simulink model "ai_layered_control_bench"  (R2024b)
settings: Solver=ode1  StartTime=0.0  StopTime=40  FixedStep=0.001  RelTol=1e-3
settings Model: Creator=ai-layered-control  LastModifiedBy=xiaol

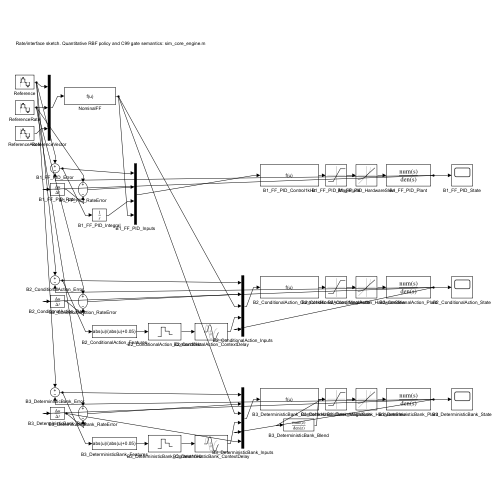
[thumbnail: Simulink's stored preview of the top-level diagram]
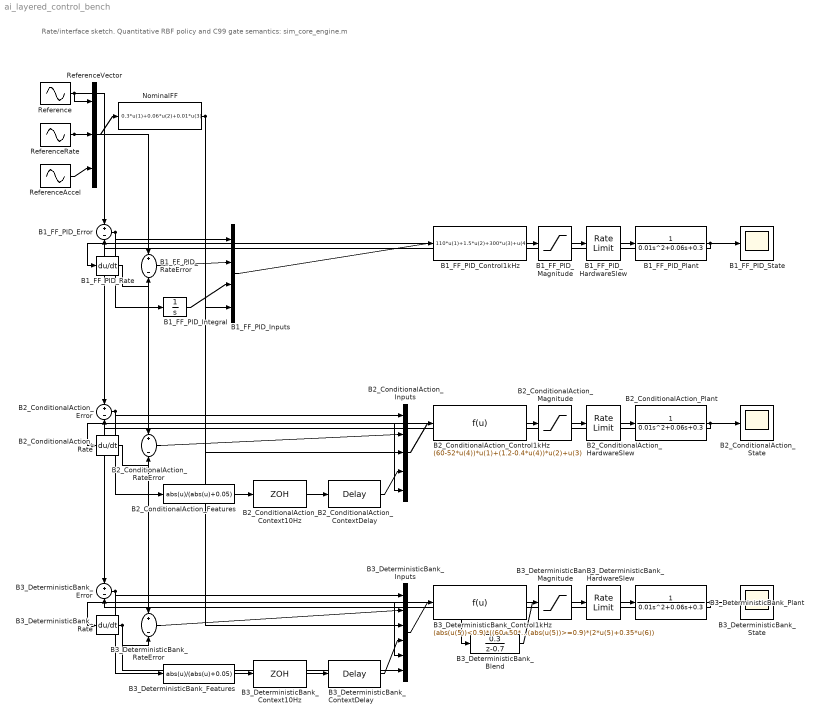
== system ai_layered_control_bench ==
  note: Rate/interface sketch. Quantitative RBF policy and C99 gate semantics: sim_core_engine.m
  B1_FF_PID_Control1kHz : Fcn  Expr=110*u(1)+1.5*u(2)+300*u(3)+u(4)
  B1_FF_PID_Error : Sum  Inputs=+-
  B1_FF_PID_HardwareSlew : RateLimiter  RisingSlewLimit=2000  FallingSlewLimit=-2000  SampleTimeMode=inherited
  B1_FF_PID_Inputs : Mux
  B1_FF_PID_Integral : Integrator
  B1_FF_PID_Magnitude : Saturate  UpperLimit=20  LowerLimit=-20
  B1_FF_PID_Plant : TransferFcn  Denominator=[0.01 0.06 0.3]
  B1_FF_PID_Rate : Derivative
  B1_FF_PID_RateError : Sum  Inputs=+-
  B1_FF_PID_State : Scope
  B2_ConditionalAction_Context10Hz : ZeroOrderHold  SampleTime=0.1
  B2_ConditionalAction_ContextDelay : TransportDelay  DelayTime=0.1
  B2_ConditionalAction_Control1kHz : Fcn  Expr=(60-52*u(4))*u(1)+(1.2-0.4*u(4))*u(2)+u(3)
  B2_ConditionalAction_Error : Sum  Inputs=+-
  B2_ConditionalAction_Features : Fcn  Expr=abs(u)/(abs(u)+0.05)
  B2_ConditionalAction_HardwareSlew : RateLimiter  RisingSlewLimit=2000  FallingSlewLimit=-2000  SampleTimeMode=inherited
  B2_ConditionalAction_Inputs : Mux  Inputs=5
  B2_ConditionalAction_Magnitude : Saturate  UpperLimit=20  LowerLimit=-20
  B2_ConditionalAction_Plant : TransferFcn  Denominator=[0.01 0.06 0.3]
  B2_ConditionalAction_Rate : Derivative
  B2_ConditionalAction_RateError : Sum  Inputs=+-
  B2_ConditionalAction_State : Scope
  B3_DeterministicBank_Blend : DiscreteTransferFcn  Numerator=[0.3]  Denominator=[1 -0.7]  SampleTime=0.001
  B3_DeterministicBank_Context10Hz : ZeroOrderHold  SampleTime=0.1
  B3_DeterministicBank_ContextDelay : TransportDelay  DelayTime=0.1
  B3_DeterministicBank_Control1kHz : Fcn  Expr=(abs(u(5))<0.9)*((60+50*(u(4)>0.5))*u(1)+1.2*u(2)+u(3))-(abs(u(5))>=0.9)*(2*u(5)+0.35*u(6))
  B3_DeterministicBank_Error : Sum  Inputs=+-
  B3_DeterministicBank_Features : Fcn  Expr=abs(u)/(abs(u)+0.05)
  B3_DeterministicBank_HardwareSlew : RateLimiter  RisingSlewLimit=2000  FallingSlewLimit=-2000  SampleTimeMode=inherited
  B3_DeterministicBank_Inputs : Mux  Inputs=6
  B3_DeterministicBank_Magnitude : Saturate  UpperLimit=20  LowerLimit=-20
  B3_DeterministicBank_Plant : TransferFcn  Denominator=[0.01 0.06 0.3]
  B3_DeterministicBank_Rate : Derivative
  B3_DeterministicBank_RateError : Sum  Inputs=+-
  B3_DeterministicBank_State : Scope
  NominalFF : Fcn  Expr=0.3*u(1)+0.06*u(2)+0.01*u(3)
  Reference : Sin  Amplitude=0.5  Frequency=pi  SampleTime=0.001
  ReferenceAccel : Sin  Amplitude=-0.5*pi*pi  Frequency=pi  SampleTime=0.001
  ReferenceRate : Sin  Amplitude=0.5*pi  Frequency=pi  Phase=pi/2  SampleTime=0.001
  ReferenceVector : Mux  Inputs=3
  wires:
  Reference/1 -> ReferenceVector/1, B1_FF_PID_Error/1, B2_ConditionalAction_Error/1, B3_DeterministicBank_Error/1
  ReferenceRate/1 -> ReferenceVector/2, B1_FF_PID_RateError/1, B2_ConditionalAction_RateError/1, B3_DeterministicBank_RateError/1
  ReferenceAccel/1 -> ReferenceVector/3
  ReferenceVector/1 -> NominalFF/1
  B1_FF_PID_Plant/1 -> B1_FF_PID_Error/2, B1_FF_PID_Rate/1, B1_FF_PID_State/1
  B1_FF_PID_Rate/1 -> B1_FF_PID_RateError/2
  B1_FF_PID_Error/1 -> B1_FF_PID_Integral/1, B1_FF_PID_Inputs/1
  B1_FF_PID_RateError/1 -> B1_FF_PID_Inputs/2
  B1_FF_PID_Integral/1 -> B1_FF_PID_Inputs/3
  NominalFF/1 -> B1_FF_PID_Inputs/4, B2_ConditionalAction_Inputs/3, B3_DeterministicBank_Inputs/3
  B1_FF_PID_Inputs/1 -> B1_FF_PID_Control1kHz/1
  B1_FF_PID_Control1kHz/1 -> B1_FF_PID_Magnitude/1
  B1_FF_PID_Magnitude/1 -> B1_FF_PID_HardwareSlew/1
  B1_FF_PID_HardwareSlew/1 -> B1_FF_PID_Plant/1
  B2_ConditionalAction_Plant/1 -> B2_ConditionalAction_Error/2, B2_ConditionalAction_Rate/1, B2_ConditionalAction_Inputs/5, B2_ConditionalAction_State/1
  B2_ConditionalAction_Rate/1 -> B2_ConditionalAction_RateError/2
  B2_ConditionalAction_Error/1 -> B2_ConditionalAction_Features/1, B2_ConditionalAction_Inputs/1
  B2_ConditionalAction_Features/1 -> B2_ConditionalAction_Context10Hz/1
  B2_ConditionalAction_Context10Hz/1 -> B2_ConditionalAction_ContextDelay/1
  B2_ConditionalAction_RateError/1 -> B2_ConditionalAction_Inputs/2
  B2_ConditionalAction_ContextDelay/1 -> B2_ConditionalAction_Inputs/4
  B2_ConditionalAction_Inputs/1 -> B2_ConditionalAction_Control1kHz/1
  B2_ConditionalAction_Control1kHz/1 -> B2_ConditionalAction_Magnitude/1
  B2_ConditionalAction_Magnitude/1 -> B2_ConditionalAction_HardwareSlew/1
  B2_ConditionalAction_HardwareSlew/1 -> B2_ConditionalAction_Plant/1
  B3_DeterministicBank_Plant/1 -> B3_DeterministicBank_Error/2, B3_DeterministicBank_Rate/1, B3_DeterministicBank_Inputs/5, B3_DeterministicBank_State/1
  B3_DeterministicBank_Rate/1 -> B3_DeterministicBank_RateError/2, B3_DeterministicBank_Inputs/6
  B3_DeterministicBank_Error/1 -> B3_DeterministicBank_Features/1, B3_DeterministicBank_Inputs/1
  B3_DeterministicBank_Features/1 -> B3_DeterministicBank_Context10Hz/1
  B3_DeterministicBank_Context10Hz/1 -> B3_DeterministicBank_ContextDelay/1
  B3_DeterministicBank_RateError/1 -> B3_DeterministicBank_Inputs/2
  B3_DeterministicBank_ContextDelay/1 -> B3_DeterministicBank_Inputs/4
  B3_DeterministicBank_Inputs/1 -> B3_DeterministicBank_Control1kHz/1
  B3_DeterministicBank_Control1kHz/1 -> B3_DeterministicBank_Blend/1
  B3_DeterministicBank_Blend/1 -> B3_DeterministicBank_Magnitude/1
  B3_DeterministicBank_Magnitude/1 -> B3_DeterministicBank_HardwareSlew/1
  B3_DeterministicBank_HardwareSlew/1 -> B3_DeterministicBank_Plant/1
